simulink model "EMT"  (R2024b)
settings: Solver=ode5  StartTime=0.0  StopTime=1500  FixedStep=0.002  RelTol=1e-3
PreLoadFcn:
  | parameter;
InitFcn:
  | parameter;
StopFcn:
  | save('result.mat');
values from neighbouring files (symbols this model uses):
  A = 7.3    [parameter.m]
  a11 = (1+k1)*(1+k2)/k1/k2/iq    (= 1.54241568346)    [parameter.m]
  a11_L = a11    (= 1.54241568346)    [parameter.m]
  a12 = -(1+k1+k2)*(1+k3)/k1/k2    (= -3.86074191629)    [parameter.m]
  a12_L = a11*(1+k3+k4)/(1+k3)    (= 2.43173643789)    [parameter.m]
  a21 = -(1+k2)/k1/iq    (= -1.04963112005)    [parameter.m]
  a22 = (1+k1+k2)/k1    (= 2.46948356808)    [parameter.m]
  B = 2.71    [parameter.m]
  b11 = 0    [parameter.m]
  b12 = (1+k3)    (= 3.33)    [parameter.m]
  b21 = (1+k2)/iq    (= 2.23571428571)    [parameter.m]
  b22 = -k2    (= -2.13)    [parameter.m]
  C1_shift = 200    [parameter.m]
  Cb = 70    [parameter.m]
  Cd = 0.6    [parameter.m]
  eff_generator = eff_motor    [parameter.m]
  eff_motor = [0.80 0.80 0.84 0.84 0.83 0.85 0.83 0.83 0.83 0.80 0.80 0.80 ... (first row only)    [parameter.m]
  ele_map = [10.00,11.46,14.13,19.24,20.94,23.21,20.29,20.23,22.28,17.66,16.24,18.95,20.79,16.98,18.22,16.52,18.29,20.67,20.82,23.14,23.36,21.30,17.71,20.26,19.53,21.18,23.13,22.79,19.35,16.77,20.50,19.02,20.56,21.90,23.91,20.40,18.45,22.70,22.38,22.48,21.84,17.76,20.13,22.61,19.35,19.36,21.56,20.37,18.38,17.96,18.38,17.24,18.99,22.31,23.50,18.24,22.11,20.73,20.35,18.91,22.88,20.92,18.75,16.85,21.94,17.80,19. ...(+2007 chars)    [parameter.m]
  Fb_max = 5.5*mass    (= 247500)    [parameter.m]
  ic = 4.42    [parameter.m]
  JA = 0.4    [parameter.m]
  JB = JA    (= 0.4)    [parameter.m]
  Jc3r4 = 1e-2    (= 0.01)    [parameter.m]
  Je = 2.5    [parameter.m]
  Jh = 1e-2    (= 0.01)    [parameter.m]
  kh = 2.88    [parameter.m]
  kt = 1.83    [parameter.m]
  L = 4.472    [parameter.m]
  mass = 45000    [parameter.m]
  miu_max = 0.8    [parameter.m]
  n_generator = n_motor    [parameter.m]
  n_motor = [0 0.1 0.25 0.4 0.55 0.7 0.85 1 1.15 1.3 1.45 2.2]*3185    [parameter.m]
  nA_map = [-6000:50:-3250 -3200 0 3200 3250:50:6000]    [parameter.m]    (also in plot_result.m = [-7000:50:-3250 -3200 0 3200 3250:50:7000])
  nA_max = max(nA_map)    [parameter.m]
  nA_min = min(nA_map)    [parameter.m]
  nB_map = nA_map    [parameter.m]    (also in plot_result.m = [-7000:50:-3250 -3200 0 3200 3250:50:7000])
  nB_max = nA_max    [parameter.m]
  nB_min = nA_min    [parameter.m]
  ne_idl = 3000    [parameter.m]
  ne_map = [1600,1700,1800,1900,2000,2100,2200,2300,2400,2500,2600,2700,2800,2900,3000,3100,3200,3300,3400,3500,3600,3700,3800,3900,4000,4100,4200,4500]    [parameter.m]
  ne_max = 4200    [parameter.m]
  ne_min = 1600    [parameter.m]
  ne_start = 200    [parameter.m]
  nZ_map = [-8000:50:-4850 -4800 0 4800 4850:50:8000]    [parameter.m]
  Pb_epr = [-45 -45 -40 -30 0 30 40 45 45]    [parameter.m]
  Pb_max = [0 40 45 45 45]    [parameter.m]
  Pb_min = [-45 -45 -45 -40 0]    [parameter.m]
  Pe_ass = 210+20    (= 230)    [parameter.m]
  Pe_max = 1103    [parameter.m]
  PN0 = 0    [parameter.m]
  R_map = [0.90 0.89 0.90 0.91 0.92 0.93 0.94 0.95 0.96 0.97 0.98]/10    [parameter.m]
  rz = 0.318    [parameter.m]
  SOC0 = 60    [parameter.m]
  SOC_epr = [30 31 50 59 60 61 70 79 80]    [parameter.m]
  SOC_map = 0:10:100    [parameter.m]
  T_generator = T_motor    [parameter.m]
  T_motor = [0 0.3 0.8 1.3 1.8 2.3 2.8]/1.8*1110    [parameter.m]
  TA_max_map = [370*9549./(6000:-50:3250) 1110 1110 1110 370*9549./(3250:50:6000)]    [parameter.m]    (also in plot_result.m = [370*9549./(7000:-50:3250) 1100 1100 1100 370*9549./(3250:50)
  TA_min_map = -TA_max_map    [parameter.m]
  TAf = 0    [parameter.m]
  TB_max_map = TA_max_map    [parameter.m]    (also in plot_result.m = [370*9549./(7000:-50:3250) 1110 1110 1110 370*9549./(3250:50)
  TB_min_map = TA_min_map    [parameter.m]
  TBf = TAf    (= 0)    [parameter.m]
  Te_map = [0,599,798,998,1168,1324,1495,1660,1822,1970,2106,2235,2355,2458,2508,2543,2565,2606,2613,2649,2658,2689,2701,2707,2719,2724,2728,2740,2743,2754]    [parameter.m]
  Te_max_map = [1168,1324,1495,1660,1822,1970,2106,2235,2355,2458,2543,2606,2658,2701,2728,2743,2754,2743,2740,2724,2719,2707,2689,2649,2613,2565,2508,998]    [parameter.m]
  Te_start = 1600    [parameter.m]
  Tef = 100    [parameter.m]
  Time = 0:0.1:200    [parameter.m]
  Time_ele = 0:4:1600    [parameter.m]
  TS_A = 0.2    [parameter.m]
  TS_B = TS_A    (= 0.2)    [parameter.m]
  TS_C0 = 0.2    [parameter.m]
  TS_C1 = 0.2    [parameter.m]
  Ts_e = 0.1    [parameter.m]
  TS_Z1 = 0.2    [parameter.m]
  TS_Z2 = 0.2    [parameter.m]
  TZ_max_map = [450*9549./(8000:-50:4850) 1000 1000 1000 450*9549./(4850:50:8000)]    [parameter.m]
  TZ_min_map = -TZ_max_map    [parameter.m]
  Uoc_map = [3.258,3.668,3.733,3.783,3.833,3.877,3.912,3.941,3.973,4.013,4.200]*250    [parameter.m]
  v_cyc = 0.*(0<=Time&Time<11)+(3.75.*Time-41.25).*(11<=Time&Time<15)+15.*(15<=Time&Time<23)+(-3.*Time+84).*(23<=Time&Time<28)+0.*(28<=Time&Time<49)+(8.*Time/3-392/3).*(49<=Time&Time<61)+32.*(61<=Time&Time<85)+(-32.*Time/11+3072/11).*(85<=Time&Time<96)+0.*(96<=Time&Time<117)+(25.*Time/13-2925/13).*(117<=Time&Time<143)+50.*(143<=Time&Time<155)+(-15.*Time/8+2725/8).*(155<=Time&Time<163)+35.*(163<=Time&Time<17 ...(+70 chars)    [parameter.m]
  V_Shift12 = 32    [parameter.m]
  V_Shift21 = 25    [parameter.m]
  Voltage_epr = [750 760 900 1000 1050]    [parameter.m]
  Y_engine = 0.955    [parameter.m]
  Yc = 0.98    [parameter.m]
  Yh = 0.96    [parameter.m]
  Z1_shift = 200    [parameter.m]
  Z2_shift = 200    [parameter.m]
undefined symbols (not defined in the file or in its folder): sigbuilder_block
libraries: fl_lib x82, nesl_utility x55, simulink x49, sdl_lib x10, simulink_need_slupdate x6, powerlib_extras x1
(part 2 of 6)

== system EMT/Control Unit/Control/Stage Judge ==
  Add : Sum  Inputs=++++
  EVT1_H Stage : Subsystem
  EVT2 Stage : Subsystem
  Prepare Stage : Subsystem
  Shift Stage : Subsystem
  stage : Outport
  tag scope: stage=global
  wires:
  EVT2 Stage/1(Out1) -> Add/4
  EVT1_H Stage/1(Out1) -> Add/2
  Shift Stage/1(Out1) -> Add/3
  Prepare Stage/1(Out1) -> Add/1
  Add/1 -> stage/1, [stage]

== system EMT/Control Unit/Driver/Electric Power Requirement ==
  " 0.1" : ManualSwitch  CurrentSetting=0
  1-D Lookup Table1 : Lookup_n-D  NumberOfTableDimensions=1  BreakpointsForDimension1=Time_ele  Table=ele_map  RndMeth=Simplest
  10 : ManualSwitch
  Add Power : ManualSwitch
  Clock1 : Clock
  ElectricPower : Display
  Saturation : Saturate  UpperLimit=300  LowerLimit=0
  Sub Power : ManualSwitch  CurrentSetting=0
  Subsystem4 : Subsystem  mask{Parameter1=on}
      mask prompts: Parameter1 "Pedal"
  Subsystem6 : Subsystem
  Transfer Fcn1 : TransferFcn  Denominator=[0.02 1]
  tag scope: ElectricPower=global
  wires:
  Subsystem4/1(Out1) -> Add Power/1
  Subsystem4/2(Out2) -> Add Power/2
  Subsystem4/3(Out3) -> Sub Power/1
  Add Power/1 -> Subsystem6/1(Add)
  Sub Power/1 -> Subsystem6/2(Sub)
  Subsystem4/4(Out4) -> Sub Power/2
  Subsystem4/5(Out5) -> " 0.1"/1
  Subsystem4/6(Out6) -> " 0.1"/2
  Subsystem4/7(Out7) -> 10/1
  Subsystem4/8(Out8) -> 10/2
  " 0.1"/1 -> Subsystem6/3(0.1)
  10/1 -> Subsystem6/4(10)
  Clock1/1 -> 1-D Lookup Table1/1
  Transfer Fcn1/1 -> [ElectricPower], ElectricPower/1
  Saturation/1 -> Transfer Fcn1/1
  1-D Lookup Table1/1 -> Saturation/1

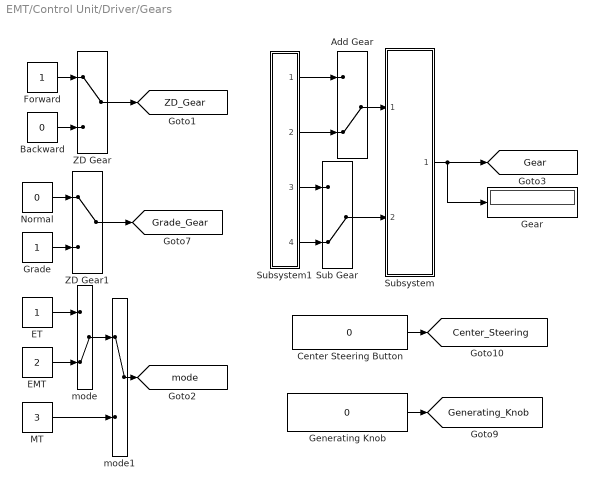
== system EMT/Control Unit/Driver/Gears ==
  "Add Gear " : ManualSwitch  CurrentSetting=0
  Backward : Constant  Value=0
  Center Steering Button : Constant  Value=0
  EMT : Constant  Value=2
  ET : Constant
  Forward : Constant
  Gear : Display
  Generating Knob : Constant  Value=0
  Grade : Constant
  MT : Constant  Value=3
  Normal : Constant  Value=0
  Sub Gear : ManualSwitch  CurrentSetting=0
  Subsystem : Subsystem
  Subsystem1 : Subsystem
  ZD Gear : ManualSwitch
  ZD Gear1 : ManualSwitch
  mode : ManualSwitch  CurrentSetting=0
  mode1 : ManualSwitch
  tag scope: Center_Steering=global, Gear=global, Generating_Knob=global, Grade_Gear=global, ZD_Gear=global, mode=global
  wires:
  ZD Gear1/1 -> [Grade_Gear]
  Normal/1 -> ZD Gear1/1
  Grade/1 -> ZD Gear1/2
  Center Steering Button/1 -> [Center_Steering]
  Generating Knob/1 -> [Generating_Knob]
  mode/1 -> mode1/1
  mode1/1 -> [mode]
  MT/1 -> mode1/2
  EMT/1 -> mode/2
  Subsystem/1(Gear) -> [Gear], Gear/1
  Sub Gear/1 -> Subsystem/2(Sub)
  "Add Gear "/1 -> Subsystem/1(Add)
  Subsystem1/4(4) -> Sub Gear/2
  Subsystem1/3(3) -> Sub Gear/1
  Subsystem1/2(2) -> "Add Gear "/2
  Subsystem1/1(1) -> "Add Gear "/1
  ET/1 -> mode/1
  ZD Gear/1 -> [ZD_Gear]
  Forward/1 -> ZD Gear/1
  Backward/1 -> ZD Gear/2

== system EMT/Control Unit/Driver/Grade Angle ==
  " 0.1" : ManualSwitch  CurrentSetting=0
  10 : ManualSwitch
  Add angle : ManualSwitch
  Forward : Constant  Value=32
  Forward1 : Constant  Value=0
  Sub angle : ManualSwitch  CurrentSetting=0
  Subsystem4 : Subsystem  mask{Parameter1=on}
      mask prompts: Parameter1 "Pedal"
  Subsystem6 : Subsystem
  Transfer Fcn1 : TransferFcn  Denominator=[0.02 1]
  angle : Display
  tag scope: angle=global
  wires:
  Subsystem4/1(Out1) -> Add angle/1
  Subsystem4/2(Out2) -> Add angle/2
  Subsystem4/3(Out3) -> Sub angle/1
  Add angle/1 -> Subsystem6/1(Add)
  Sub angle/1 -> Subsystem6/2(Sub)
  Subsystem4/4(Out4) -> Sub angle/2
  Subsystem4/5(Out5) -> " 0.1"/1
  Subsystem4/6(Out6) -> " 0.1"/2
  Subsystem4/7(Out7) -> 10/1
  Subsystem4/8(Out8) -> 10/2
  " 0.1"/1 -> Subsystem6/3(0.1)
  10/1 -> Subsystem6/4(10)
  Subsystem6/1(angle) -> Transfer Fcn1/1, angle/1
  Forward1/1 -> [angle]

== system EMT/Control Unit/Driver/Ground Resistance Coefficient ==
  *0.1 : ManualSwitch
  *10 : ManualSwitch
  Add : Sum
  Add fg : ManualSwitch  CurrentSetting=0
  Add1 : Sum
  Forward : Constant  Value=0.07
  Forward1 : Constant  Value=0.045
  Road : Subsystem
  Road1 : Subsystem
  Saturation : Saturate  UpperLimit=0.6  LowerLimit=0.04
  Saturation1 : Saturate  UpperLimit=0.6  LowerLimit=0.04
  Sub fg : ManualSwitch  CurrentSetting=0
  Subsystem2 : Subsystem  mask{Parameter1=on}
      mask prompts: Parameter1 "Pedal"
  Subsystem3 : Subsystem
  Transfer Fcn1 : TransferFcn  Denominator=[0.02 1]
  Uniform Random Number : UniformRandomNumber  Minimum=-0.01  Maximum=0.01  SampleTime=1
  fg : Display
  tag scope: fg_act=global
  wires:
  Road/1(fg) -> Add/2
  Subsystem3/1(fg) -> Add/1
  Subsystem2/1(Out1) -> Add fg/1
  Subsystem2/2(Out2) -> Add fg/2
  Subsystem2/3(Out3) -> Sub fg/1
  Add fg/1 -> Subsystem3/1(Add)
  Sub fg/1 -> Subsystem3/2(Sub)
  Subsystem2/4(Out4) -> Sub fg/2
  Subsystem2/5(Out5) -> *0.1/1
  Subsystem2/6(Out6) -> *0.1/2
  Subsystem2/7(Out7) -> *10/1
  Subsystem2/8(Out8) -> *10/2
  *0.1/1 -> Subsystem3/3(0.1)
  *10/1 -> Subsystem3/4(10)
  Transfer Fcn1/1 -> fg/1
  Add/1 -> Saturation/1
  Uniform Random Number/1 -> Add1/2
  Road1/1(fg) -> Saturation1/1
  Forward/1 -> Add1/1
  Add1/1 -> Transfer Fcn1/1
  Forward1/1 -> [fg_act]

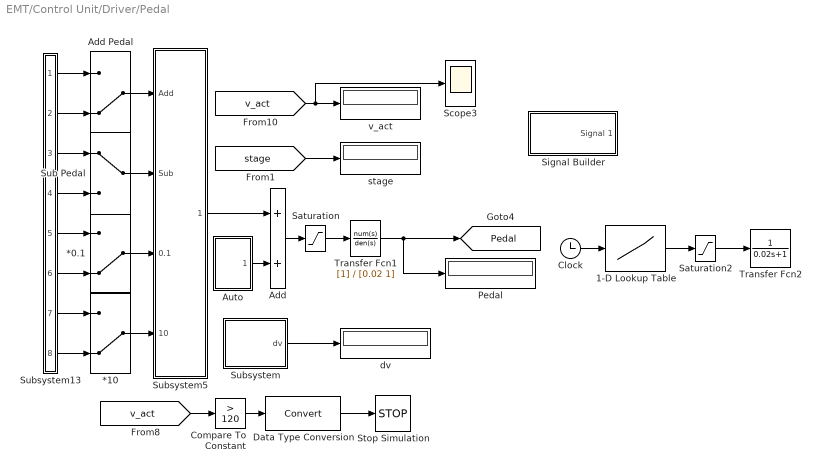
== system EMT/Control Unit/Driver/Pedal  ==
  *0.1 : ManualSwitch  CurrentSetting=0
  *10 : ManualSwitch  CurrentSetting=0
  1-D Lookup Table : Lookup_n-D  NumberOfTableDimensions=1  BreakpointsForDimension1=[0 100 101 200]  Table=[1 1 -1 -1]  RndMeth=Simplest
  Add : Sum
  Add Pedal : ManualSwitch  CurrentSetting=0
  Auto : Subsystem
  Clock : Clock
  Compare To Constant : simulink/Logic and Bit Operations/Compare To Constant  relop=>  const=120  OutDataTypeStr=uint8
  Data Type Conversion : DataTypeConversion  SaturateOnIntegerOverflow=off  RndMeth=Floor
  Pedal : Display
  Saturation : Saturate  UpperLimit=1  LowerLimit=-1
  Saturation2 : Saturate  UpperLimit=1  LowerLimit=-1
  Scope3 : Scope
  Signal Builder : Subsystem  Tag=STV Subsys  LoadFcn=sigbuilder_block('load');  StartFcn=sigbuilder_block('start');  StopFcn=sigbuilder_block('stop');  ClipboardFcn=sigbuilder_block('clipboard');  mask(Sigbuilder block){tuvar=[0:10]}
      mask help: Simulink:masks:SigbuilderBlock_MD
      mask init:
      | if ~strcmp(get_param(bdroot(gcbh),'SimulationStatus'),'stopped') tuvar = sigbuilder_block('maskInit'); end
      settings: CopyFcn=sigbuilder_block('copy');  DeleteFcn=sigbuilder_block('delete');  ModelCloseFcn=sigbuilder_block('modelClose');  PreSaveFcn=sigbuilder_block('preSave');  PauseFcn=sigbuilder_block('pause')  ContinueFcn=sigbuilder_block('continue')  NameChangeFcn=sigbuilder_block('namechange');  OpenFcn=sigbuilder_block('open',[437.25 199.5 550.5 399.75 ]);  CloseFcn=sigbuilder_block('close');
      mask Display: plot(0, 0, 100, 100,[2, 2, 32, 32, 2], [68, 8, 8, 68, 68],[32, 2], [38, 38], [32, 19, 2],[53, 60, 44], [32, 17, 17, 2],[16, 16, 31, 31]);txt = getActiveGroup(gcbh);text(2, 100, txt,'verticalAlignment', 'top');
  Stop Simulation : Stop
  Sub Pedal : ManualSwitch
  Subsystem : Subsystem
  Subsystem13 : Subsystem  mask{Parameter1=on}
      mask prompts: Parameter1 "Pedal"
  Subsystem5 : Subsystem
  Transfer Fcn1 : TransferFcn  Denominator=[0.02 1]
  Transfer Fcn2 : TransferFcn  Denominator=[0.02 1]
  dv : Display
  stage : Display
  v_act : Display
  tag scope: Pedal=global
  wires:
  Subsystem5/1(Pedal) -> Add/1
  Subsystem/1(dv) -> dv/1
  [stage] -> stage/1
  [v_act] -> Scope3/1, v_act/1
  *10/1 -> Subsystem5/4(10)
  *0.1/1 -> Subsystem5/3(0.1)
  Subsystem13/8(Out8) -> *10/2
  Subsystem13/7(Out7) -> *10/1
  Subsystem13/6(Out6) -> *0.1/2
  Subsystem13/5(Out5) -> *0.1/1
  Subsystem13/4(Out4) -> Sub Pedal/2
  Sub Pedal/1 -> Subsystem5/2(Sub)
  Add Pedal/1 -> Subsystem5/1(Add)
  Subsystem13/3(Out3) -> Sub Pedal/1
  Subsystem13/2(Out2) -> Add Pedal/2
  Subsystem13/1(Out1) -> Add Pedal/1
  [v_act] -> Compare To Constant/1
  Compare To Constant/1 -> Data Type Conversion/1
  Data Type Conversion/1 -> Stop Simulation/1
  Saturation/1 -> Transfer Fcn1/1
  Add/1 -> Saturation/1
  Clock/1 -> 1-D Lookup Table/1
  1-D Lookup Table/1 -> Saturation2/1
  Saturation2/1 -> Transfer Fcn2/1
  Auto/1(Pedal) -> Add/2
  Transfer Fcn1/1 -> Pedal/1, [Pedal]

== system EMT/Control Unit/Driver/Wheel Angle ==
  " x 0.1" : ManualSwitch  CurrentSetting=0
  Add wheel : ManualSwitch
  Sub Wheel : ManualSwitch  CurrentSetting=0
  Subsystem1 : Subsystem  mask{Parameter1=on}
      mask prompts: Parameter1 "Pedal"
  Subsystem2 : Subsystem
  Wheel : Display
  x10 : ManualSwitch
  tag scope: Wheel=global
  wires:
  Subsystem2/1(wheel) -> Wheel/1, [Wheel]
  Subsystem1/1(Out1) -> Add wheel/1
  Subsystem1/2(Out2) -> Add wheel/2
  Subsystem1/3(Out3) -> Sub Wheel/1
  Add wheel/1 -> Subsystem2/1(Add)
  Sub Wheel/1 -> Subsystem2/2(Sub)
  Subsystem1/4(Out4) -> Sub Wheel/2
  Subsystem1/5(Out5) -> " x 0.1"/1
  Subsystem1/6(Out6) -> " x 0.1"/2
  Subsystem1/7(Out7) -> x10/1
  Subsystem1/8(Out8) -> x10/2
  " x 0.1"/1 -> Subsystem2/3(0.1)
  x10/1 -> Subsystem2/4(10)

== system EMT/Front Gear/C0/C0 ==
  Press : Inport
  C0 : sdl_lib/Clutches/Disc Friction Clutch  geometry_model=2  r_eff=130 mm  d_o=145*2 mm  d_i=110*2 mm  nS=6  piston_area=0.0347 m^2  unidirectional=0  friction_model=1  mu_w_vector=[ 0 0.1 0.2 0.3 0.4 0.5 1 2 5 10 100 1000 ] rad/s  temperature_TLU=[280.0, 300.0, 320.0] K  mu_static=0.10  mu_static_vector=[0.4, 0.38, 0.36]  mu_coulomb=0.06  mu_coulomb_vector=[ 0.29 0.28 0.26 0.22 0.21 0.2 0.2 0.19 0.19 0.19 0.19 0.19 ]  mu_coulomb_temp_vector=[0.3, 0.28, 0.25]  mu_coulomb_matrix=[0.34, 0.32, 0.3; 0.3, 0.28, 0.25; 0.25, 0.2, 0.15]  mu_interp_method=1  mu_extrap_method=1  d_f=0.6  w_tol=0.001 rad/s  pressure_min=1560 Pa  mu_visc=0.0256 N*m/(rad/s)  initial_state_locked=1  thermal_mass=25 kJ/K  T_init=300 K
      settings: InternalSimscapePortConfiguration="{\"Bottom\":[],\"Left\":[{\"id\":\"P\",\"label\":\"P\",\"type\":\"input\"},{\"id\":\"B\",\"label\":\"B\",\"type\":\"foundation.mechanical.rotational.rotational\"}],\"Right\":[{\"id\":\"F\",\"label\":\"F\",\"type\":\"foundation.mechanical.rotational.rotational\"}],\"Top\":[]}"
  Simulink-PS Converter : nesl_utility/Simulink-PS Converter  PhysicalDomain=network_engine_domain  SubClassName=ps_input  LeftPortType=input  RightPortType=output  PseudoPeriodic=off  Frequencies=[]  NoiseDistribution=none  NoiseParameters=[]  Unit=Pa  AffineConversion=off  FilteringAndDerivatives=filter  SimscapeFilterOrder=1  InputFilterTimeConstant=.001  UdotUserProvided=1
  Slip Sensor : Subsystem  mask(Slip Sensor){}
      mask help: The speed unit is r/min.
  Tire Radius2 : Gain  Gain=2500000
  In : PMIOPort  Side=Left
  Out : PMIOPort  Port=2  Side=Right
  r/min : Outport
  wires:
  Slip Sensor/1(r/min) -> r/min/1
  Press/1 -> Tire Radius2/1
  Tire Radius2/1 -> Simulink-PS Converter/1
  connections:
  Slip Sensor/LConn1 -- C0/LConn2 -- In/RConn1
  Slip Sensor/RConn1 -- C0/RConn1 -- Out/RConn1
  Simulink-PS Converter/RConn1 -- C0/LConn1

== system EMT/Front Gear/C0/Power ==
  Gain1 : Gain  Gain=1/9549
  Product3 : Product  RndMeth=Zero
  Speed Sensor : Subsystem  mask(Speed Sensor){}
      mask help: The speed unit is r/min.
  Torque Sensor : Subsystem  mask(Torque Sensor){}
      mask help: The torque unit is Nm.
  In : PMIOPort  Side=Left
  Out : PMIOPort  Port=2  Side=Right
  kW : Outport
  wires:
  Speed Sensor/1(r/min) -> Product3/2
  Torque Sensor/1(Nm) -> Gain1/1
  Gain1/1 -> Product3/1
  Product3/1 -> kW/1
  connections:
  Out/RConn1 -- Torque Sensor/RConn1 -- Speed Sensor/LConn1
  In/RConn1 -- Torque Sensor/LConn1

== system EMT/Front Gear/C0/Power1 ==
  Gain1 : Gain  Gain=1/9549
  Product3 : Product  RndMeth=Zero
  Speed Sensor : Subsystem  mask(Speed Sensor){}
      mask help: The speed unit is r/min.
  Torque Sensor : Subsystem  mask(Torque Sensor){}
      mask help: The torque unit is Nm.
  In : PMIOPort  Side=Left
  Out : PMIOPort  Port=2  Side=Right
  kW : Outport
  wires:
  Product3/1 -> kW/1
  Gain1/1 -> Product3/1
  Torque Sensor/1(Nm) -> Gain1/1
  Speed Sensor/1(r/min) -> Product3/2
  connections:
  In/RConn1 -- Torque Sensor/LConn1
  Torque Sensor/RConn1 -- Out/RConn1 -- Speed Sensor/LConn1

== system EMT/Front Gear/Subsystem/Speed Sensor ==
  Ideal Rotational Motion Sensor : fl_lib/Mechanical/Mechanical Sensors/Ideal Rotational Motion Sensor  reference=foundation.enum.MeasurementReference.difference  acceleration_port=false  velocity_port=true  position_port=true  wrap_angle=false  offset=0 rad
  PS-Simulink Converter : nesl_utility/PS-Simulink Converter  PhysicalDomain=network_engine_domain  SubClassName=ps_output  LeftPortType=input  RightPortType=output  PseudoPeriodic=off  Frequencies=[]  VectorFormat=1-D array  Unit=rad/s  AffineConversion=off
  Reference : fl_lib/Mechanical/Rotational Elements/Mechanical Rotational Reference
  Tire Radius2 : Gain  Gain=30/pi
  shaft : PMIOPort  Side=Left
  r/min : Outport
  wires:
  Tire Radius2/1 -> r/min/1
  PS-Simulink Converter/1 -> Tire Radius2/1
  connections:
  shaft/RConn1 -- Ideal Rotational Motion Sensor/LConn1
  Reference/LConn1 -- Ideal Rotational Motion Sensor/RConn1
  PS-Simulink Converter/LConn1 -- Ideal Rotational Motion Sensor/RConn2

== system EMT/Front Gear/Subsystem/Torque Sensor ==
  Ideal Torque Sensor : fl_lib/Mechanical/Mechanical Sensors/Ideal Torque Sensor
  PS-Simulink Converter : nesl_utility/PS-Simulink Converter  PhysicalDomain=network_engine_domain  SubClassName=ps_output  LeftPortType=input  RightPortType=output  PseudoPeriodic=off  Frequencies=[]  VectorFormat=1-D array  Unit=1  AffineConversion=off
  In : PMIOPort  Side=Left
  Out : PMIOPort  Port=2  Side=Right
  Nm : Outport
  wires:
  PS-Simulink Converter/1 -> Nm/1
  connections:
  PS-Simulink Converter/LConn1 -- Ideal Torque Sensor/RConn2
  In/RConn1 -- Ideal Torque Sensor/LConn1
  Ideal Torque Sensor/RConn1 -- Out/RConn1

== system EMT/Power Coupler /C1/C2 ==
  Press : Inport
  C1 : sdl_lib/Clutches/Disc Friction Clutch  geometry_model=2  r_eff=130 mm  d_o=167*2 mm  d_i=143*2 mm  nS=8  piston_area=0.0290 m^2  unidirectional=0  friction_model=1  mu_w_vector=[ 0 0.1 0.2 0.3 0.4 0.5 1 2 5 10 100 1000 ] rad/s  temperature_TLU=[280.0, 300.0, 320.0] K  mu_static=0.10  mu_static_vector=[0.4, 0.38, 0.36]  mu_coulomb=0.06  mu_coulomb_vector=[ 0.29 0.28 0.26 0.22 0.21 0.2 0.2 0.19 0.19 0.19 0.19 0.19 ]  mu_coulomb_temp_vector=[0.3, 0.28, 0.25]  mu_coulomb_matrix=[0.34, 0.32, 0.3; 0.3, 0.28, 0.25; 0.25, 0.2, 0.15]  mu_interp_method=1  mu_extrap_method=1  d_f=0.6  w_tol=0.001 rad/s  pressure_min=1840 Pa  mu_visc=0.0414 N*m/(rad/s)  initial_state_locked=0  thermal_mass=25 kJ/K  T_init=300 K
      settings: InternalSimscapePortConfiguration="{\"Bottom\":[],\"Left\":[{\"id\":\"P\",\"label\":\"P\",\"type\":\"input\"},{\"id\":\"B\",\"label\":\"B\",\"type\":\"foundation.mechanical.rotational.rotational\"}],\"Right\":[{\"id\":\"F\",\"label\":\"F\",\"type\":\"foundation.mechanical.rotational.rotational\"}],\"Top\":[]}"
  Simulink-PS Converter : nesl_utility/Simulink-PS Converter  PhysicalDomain=network_engine_domain  SubClassName=ps_input  LeftPortType=input  RightPortType=output  PseudoPeriodic=off  Frequencies=[]  NoiseDistribution=none  NoiseParameters=[]  Unit=Pa  AffineConversion=off  FilteringAndDerivatives=filter  SimscapeFilterOrder=1  InputFilterTimeConstant=.001  UdotUserProvided=1
  Slip Sensor : Subsystem  mask(Slip Sensor){}
      mask help: The speed unit is r/min.
  Tire Radius2 : Gain  Gain=2500000
  In : PMIOPort  Side=Left
  Out : PMIOPort  Port=2  Side=Right
  r/min : Outport
  wires:
  Tire Radius2/1 -> Simulink-PS Converter/1
  Press/1 -> Tire Radius2/1
  Slip Sensor/1(r/min) -> r/min/1
  connections:
  Simulink-PS Converter/RConn1 -- C1/LConn1
  In/RConn1 -- C1/LConn2 -- Slip Sensor/LConn1
  C1/RConn1 -- Out/RConn1 -- Slip Sensor/RConn1

== system EMT/Power Coupler /C1/Power ==
  Gain1 : Gain  Gain=1/9549
  Product3 : Product  RndMeth=Zero
  Speed Sensor : Subsystem  mask(Speed Sensor){}
      mask help: The speed unit is r/min.
  Torque Sensor : Subsystem  mask(Torque Sensor){}
      mask help: The torque unit is Nm.
  In : PMIOPort  Side=Left
  Out : PMIOPort  Port=2  Side=Right
  kW : Outport
  wires:
  Product3/1 -> kW/1
  Gain1/1 -> Product3/1
  Torque Sensor/1(Nm) -> Gain1/1
  Speed Sensor/1(r/min) -> Product3/2
  connections:
  In/RConn1 -- Torque Sensor/LConn1
  Torque Sensor/RConn1 -- Out/RConn1 -- Speed Sensor/LConn1

== system EMT/Power Coupler /C1/Power1 ==
  Gain1 : Gain  Gain=1/9549
  Product3 : Product  RndMeth=Zero
  Speed Sensor : Subsystem  mask(Speed Sensor){}
      mask help: The speed unit is r/min.
  Torque Sensor : Subsystem  mask(Torque Sensor){}
      mask help: The torque unit is Nm.
  In : PMIOPort  Side=Left
  Out : PMIOPort  Port=2  Side=Right
  kW : Outport
  wires:
  Speed Sensor/1(r/min) -> Product3/2
  Torque Sensor/1(Nm) -> Gain1/1
  Gain1/1 -> Product3/1
  Product3/1 -> kW/1
  connections:
  Speed Sensor/LConn1 -- Out/RConn1 -- Torque Sensor/RConn1
  In/RConn1 -- Torque Sensor/LConn1

== system EMT/Power Coupler /Z1/Z ==
  Abs : Abs  SaturateOnIntegerOverflow=off
  Add : Sum  Inputs=+-
  Power : Subsystem
  Power1 : Subsystem
  Z1 : Subsystem
  In : PMIOPort  Side=Left
  Out : PMIOPort  Port=2  Side=Right
  tag scope: Z1_loss=global, Z1_rela=global
  wires:
  Z1/1(r/min) -> [Z1_rela]
  [Press_Z1] -> Z1/1(Press)
  Power1/1(kW) -> Add/2
  Power/1(kW) -> Add/1
  Abs/1 -> [Z1_loss]
  Add/1 -> Abs/1
  connections:
  In/RConn1 -- Power/LConn1
  Power/RConn1 -- Z1/LConn1
  Z1/RConn1 -- Power1/LConn1
  Power1/RConn1 -- Out/RConn1

== system EMT/Power Coupler /Z2/Z ==
  Abs : Abs  SaturateOnIntegerOverflow=off
  Add : Sum  Inputs=+-
  Power : Subsystem
  Power1 : Subsystem
  Z2 : Subsystem
  In : PMIOPort  Side=Left
  Out : PMIOPort  Port=2  Side=Right
  tag scope: Z2_loss=global, Z2_rela=global
  wires:
  [Press_Z2] -> Z2/1(Press)
  Z2/1(r/min) -> [Z2_rela]
  Add/1 -> Abs/1
  Abs/1 -> [Z2_loss]
  Power1/1(kW) -> Add/2
  Power/1(kW) -> Add/1
  connections:
  In/RConn1 -- Power/LConn1
  Power/RConn1 -- Z2/LConn1
  Z2/RConn1 -- Power1/LConn1
  Power1/RConn1 -- Out/RConn1

== system EMT/Rear Gear/Subsystem/Speed Sensor ==
  Ideal Rotational Motion Sensor : fl_lib/Mechanical/Mechanical Sensors/Ideal Rotational Motion Sensor  reference=foundation.enum.MeasurementReference.difference  acceleration_port=false  velocity_port=true  position_port=true  wrap_angle=false  offset=0 rad
  PS-Simulink Converter : nesl_utility/PS-Simulink Converter  PhysicalDomain=network_engine_domain  SubClassName=ps_output  LeftPortType=input  RightPortType=output  PseudoPeriodic=off  Frequencies=[]  VectorFormat=1-D array  Unit=rad/s  AffineConversion=off
  Reference : fl_lib/Mechanical/Rotational Elements/Mechanical Rotational Reference
  Tire Radius2 : Gain  Gain=30/pi
  shaft : PMIOPort  Side=Left
  r/min : Outport
  wires:
  Tire Radius2/1 -> r/min/1
  PS-Simulink Converter/1 -> Tire Radius2/1
  connections:
  shaft/RConn1 -- Ideal Rotational Motion Sensor/LConn1
  Reference/LConn1 -- Ideal Rotational Motion Sensor/RConn1
  PS-Simulink Converter/LConn1 -- Ideal Rotational Motion Sensor/RConn2

== system EMT/Rear Gear/Subsystem/Torque Sensor ==
  Ideal Torque Sensor : fl_lib/Mechanical/Mechanical Sensors/Ideal Torque Sensor
  PS-Simulink Converter : nesl_utility/PS-Simulink Converter  PhysicalDomain=network_engine_domain  SubClassName=ps_output  LeftPortType=input  RightPortType=output  PseudoPeriodic=off  Frequencies=[]  VectorFormat=1-D array  Unit=1  AffineConversion=off
  In : PMIOPort  Side=Left
  Out : PMIOPort  Port=2  Side=Right
  Nm : Outport
  wires:
  PS-Simulink Converter/1 -> Nm/1
  connections:
  PS-Simulink Converter/LConn1 -- Ideal Torque Sensor/RConn2
  In/RConn1 -- Ideal Torque Sensor/LConn1
  Ideal Torque Sensor/RConn1 -- Out/RConn1

== system EMT/Simulation Results/Engine Viewer/Fuel  ==
  FuelConsumption : Lookup2D  RowIndex=ne_map  ColumnIndex=Te_map  Table=fuel_map'  LookUpMeth=Interpolation-Use End Values  SaturateOnIntegerOverflow=off  InputSameDT=off
  Gain : Gain  Gain=1/3600/0.84/1000
  Gain1 : Gain  Gain=1/9549
  Integrator : Integrator  IgnoreLimit=on
  Product1 : Product  RndMeth=Zero
  Product2 : Product  RndMeth=Zero
  Product3 : Product  RndMeth=Zero
  Saturation : Saturate  UpperLimit=max(ne_map)  LowerLimit=min(ne_map)
  Saturation1 : Saturate  UpperLimit=max(Te_map)  LowerLimit=min(Te_map)
  Saturation2 : Saturate  UpperLimit=max(ne_map)*max(Te_map)/9549  LowerLimit=0
  fuel_L : Outport
  gpkWh : Outport  Port=2
  tag scope: eng_fuel_gpkWh=global, fuel_L=global
  wires:
  [Te_act] -> Product1/2, Saturation1/1
  [ne_act] -> Product1/1, Saturation/1
  Saturation2/1 -> Product3/2
  Gain1/1 -> Saturation2/1
  Saturation1/1 -> FuelConsumption/2
  Gain/1 -> Integrator/1
  Integrator/1 -> [fuel_L], fuel_L/1
  Product3/1 -> Gain/1
  Saturation/1 -> FuelConsumption/1
  Product1/1 -> Gain1/1
  Product2/1 -> Product3/1, [eng_fuel_gpkWh], gpkWh/1
  [engine_switch] -> Product2/1
  FuelConsumption/1 -> Product2/2

== system EMT/Simulation Results/Vehicle Viewer/Subsystem1 ==
  0 : Inport
  Constant : Constant  Value=0.001
  MinMax : MinMax  Function=max  Inputs=2
  1 : Outport
  wires:
  MinMax/1 -> 1/1
  0/1 -> MinMax/1
  Constant/1 -> MinMax/2

== system EMT/Simulation Results/Vehicle Viewer/Subsystem7 ==
  0 : Inport
  Constant : Constant  Value=0
  MinMax : MinMax  Function=max  Inputs=2
  1 : Outport
  wires:
  Constant/1 -> MinMax/2
  0/1 -> MinMax/1
  MinMax/1 -> 1/1

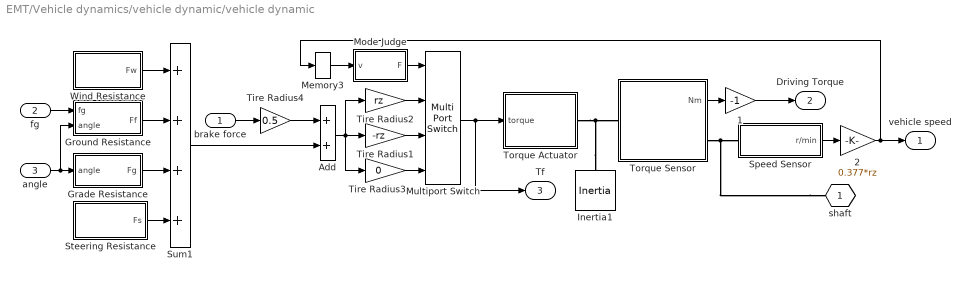
== system EMT/Vehicle dynamics/vehicle dynamic/vehicle dynamic ==
  brake force : Inport
  fg : Inport  Port=2
  angle : Inport  Port=3
  1 : Gain  Gain=-1
  2 : Gain  Gain=0.377*rz
  Add : Sum
  Grade Resistance : Subsystem
  Ground Resistance : Subsystem
  Inertia1 : fl_lib/Mechanical/Rotational Elements/Inertia  inertia=0.5*mass*rz^2 kg*m^2  num_ports=foundation.enum.numPorts2.one  w_specify=on  w_priority=High  w=0 rad/s  w_nominal_specify=off  w_nominal_value=1  w_nominal_unit=rad/s  t_specify=off  t_priority=None  t=0 N*m  t_nominal_specify=off  t_nominal_value=1  t_nominal_unit=N*m
  Memory3 : Memory
  Mode Judge : Subsystem
  Multiport Switch : MultiPortSwitch  SaturateOnIntegerOverflow=off  InputSameDT=off
  Speed Sensor : Subsystem  mask(Speed Sensor){}
      mask help: The speed unit is r/min.
  Steering Resistance : Subsystem
  Sum1 : Sum  Inputs=++++
  Tire Radius1 : Gain  Gain=-rz
  Tire Radius2 : Gain  Gain=rz
  Tire Radius3 : Gain  Gain=0
  Tire Radius4 : Gain  Gain=0.5
  Torque Actuator : Subsystem  mask(Torque Actuator){}
      mask help: The torque unit is Nm.
  Torque Sensor : Subsystem  mask(Torque Sensor){}
      mask help: The torque unit is Nm.
  Wind Resistance : Subsystem
  shaft : PMIOPort  Side=Left
  vehicle speed : Outport
  Driving Torque : Outport  Port=2
  Tf : Outport  Port=3
  wires:
  Tire Radius3/1 -> Multiport Switch/4
  Add/1 -> Tire Radius3/1, Tire Radius1/1, Tire Radius2/1
  Tire Radius1/1 -> Multiport Switch/3
  Tire Radius2/1 -> Multiport Switch/2
  Mode Judge/1(F) -> Multiport Switch/1
  1/1 -> Driving Torque/1
  Torque Sensor/1(Nm) -> 1/1
  Sum1/1 -> Add/2
  2/1 -> vehicle speed/1, Memory3/1
  brake force/1 -> Tire Radius4/1
  Speed Sensor/1(r/min) -> 2/1
  Ground Resistance/1(Ff) -> Sum1/2
  Wind Resistance/1(Fw) -> Sum1/1
  Tire Radius4/1 -> Add/1
  Steering Resistance/1(Fs) -> Sum1/4
  Grade Resistance/1(Fg) -> Sum1/3
  Memory3/1 -> Mode Judge/1(v)
  Multiport Switch/1 -> Torque Actuator/1(torque), Tf/1
  angle/1 -> Grade Resistance/1(angle), Ground Resistance/2(angle)
  fg/1 -> Ground Resistance/1(fg)
  connections:
  shaft/RConn1 -- Speed Sensor/LConn1 -- Torque Sensor/RConn1
  Inertia1/LConn1 -- Torque Actuator/RConn1 -- Torque Sensor/LConn1

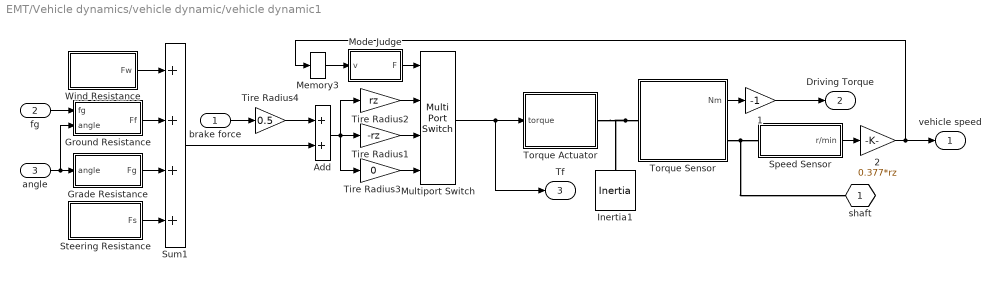
== system EMT/Vehicle dynamics/vehicle dynamic/vehicle dynamic1 ==
  brake force : Inport
  fg : Inport  Port=2
  angle : Inport  Port=3
  1 : Gain  Gain=-1
  2 : Gain  Gain=0.377*rz
  Add : Sum
  Grade Resistance : Subsystem
  Ground Resistance : Subsystem
  Inertia1 : fl_lib/Mechanical/Rotational Elements/Inertia  inertia=0.5*mass*rz^2 kg*m^2  num_ports=foundation.enum.numPorts2.one  w_specify=on  w_priority=High  w=0 rad/s  w_nominal_specify=off  w_nominal_value=1  w_nominal_unit=rad/s  t_specify=off  t_priority=None  t=0 N*m  t_nominal_specify=off  t_nominal_value=1  t_nominal_unit=N*m
  Memory3 : Memory
  Mode Judge : Subsystem
  Multiport Switch : MultiPortSwitch  SaturateOnIntegerOverflow=off  InputSameDT=off
  Speed Sensor : Subsystem  mask(Speed Sensor){}
      mask help: The speed unit is r/min.
  Steering Resistance : Subsystem
  Sum1 : Sum  Inputs=++++
  Tire Radius1 : Gain  Gain=-rz
  Tire Radius2 : Gain  Gain=rz
  Tire Radius3 : Gain  Gain=0
  Tire Radius4 : Gain  Gain=0.5
  Torque Actuator : Subsystem  mask(Torque Actuator){}
      mask help: The torque unit is Nm.
  Torque Sensor : Subsystem  mask(Torque Sensor){}
      mask help: The torque unit is Nm.
  Wind Resistance : Subsystem
  shaft : PMIOPort  Side=Left
  vehicle speed : Outport
  Driving Torque : Outport  Port=2
  Tf : Outport  Port=3
  wires:
  Memory3/1 -> Mode Judge/1(v)
  Grade Resistance/1(Fg) -> Sum1/3
  Steering Resistance/1(Fs) -> Sum1/4
  Tire Radius4/1 -> Add/1
  Wind Resistance/1(Fw) -> Sum1/1
  Ground Resistance/1(Ff) -> Sum1/2
  Speed Sensor/1(r/min) -> 2/1
  brake force/1 -> Tire Radius4/1
  2/1 -> vehicle speed/1, Memory3/1
  Sum1/1 -> Add/2
  Torque Sensor/1(Nm) -> 1/1
  1/1 -> Driving Torque/1
  Mode Judge/1(F) -> Multiport Switch/1
  Tire Radius2/1 -> Multiport Switch/2
  Tire Radius1/1 -> Multiport Switch/3
  Add/1 -> Tire Radius2/1, Tire Radius1/1, Tire Radius3/1
  Tire Radius3/1 -> Multiport Switch/4
  Multiport Switch/1 -> Torque Actuator/1(torque), Tf/1
  angle/1 -> Ground Resistance/2(angle), Grade Resistance/1(angle)
  fg/1 -> Ground Resistance/1(fg)
  connections:
  Torque Sensor/LConn1 -- Torque Actuator/RConn1 -- Inertia1/LConn1
  Torque Sensor/RConn1 -- Speed Sensor/LConn1 -- shaft/RConn1

== system EMT/engine/Engine/Speed Sensor ==
  Ideal Rotational Motion Sensor : fl_lib/Mechanical/Mechanical Sensors/Ideal Rotational Motion Sensor  reference=foundation.enum.MeasurementReference.difference  acceleration_port=false  velocity_port=true  position_port=true  wrap_angle=false  offset=0 rad
  PS-Simulink Converter : nesl_utility/PS-Simulink Converter  PhysicalDomain=network_engine_domain  SubClassName=ps_output  LeftPortType=input  RightPortType=output  PseudoPeriodic=off  Frequencies=[]  VectorFormat=1-D array  Unit=rad/s  AffineConversion=off
  Reference : fl_lib/Mechanical/Rotational Elements/Mechanical Rotational Reference
  Tire Radius2 : Gain  Gain=30/pi
  shaft : PMIOPort  Side=Left
  r/min : Outport
  wires:
  Tire Radius2/1 -> r/min/1
  PS-Simulink Converter/1 -> Tire Radius2/1
  connections:
  shaft/RConn1 -- Ideal Rotational Motion Sensor/LConn1
  Reference/LConn1 -- Ideal Rotational Motion Sensor/RConn1
  PS-Simulink Converter/LConn1 -- Ideal Rotational Motion Sensor/RConn2

== system EMT/engine/Engine/Subsystem ==
  ne_act : Inport
  Te_com : Inport  Port=2
  switch : Inport  Port=3
  Constant1 : Constant  Value=0
  Fcn : Fcn  Expr=u*(1103-180)/1103
  Lookup Table : Lookup  InputValues=ne_map  Table=Te_max_map  SaturateOnIntegerOverflow=off
  Product : Product  RndMeth=Zero
  Saturation : Saturate  UpperLimit=max(ne_map)  LowerLimit=min(ne_map)
  Saturation Dynamic : simulink/Discontinuities/Saturation Dynamic  OutMin=[]  OutMax=[]  OutDataTypeStr=Inherit: Same as second input  OutDataType=sfix(16)  OutScaling=2^-10  DoSatur=off
  Tire Radius2 : Gain  Gain=Y_engine
  Transfer Fcn1 : TransferFcn  Denominator=[T 1]
  Te_act : Outport
  Torque : Outport  Port=2
  wires:
  Transfer Fcn1/1 -> Product/1
  switch/1 -> Product/2
  Saturation Dynamic/1 -> Transfer Fcn1/1
  Saturation/1 -> Lookup Table/1
  Lookup Table/1 -> Saturation Dynamic/1
  Constant1/1 -> Saturation Dynamic/3
  Product/1 -> Tire Radius2/1, Te_act/1
  ne_act/1 -> Saturation/1
  Te_com/1 -> Saturation Dynamic/2
  Tire Radius2/1 -> Fcn/1
  Fcn/1 -> Torque/1

== system EMT/engine/Engine/Subsystem1 ==
  ne : Inport
  Abs1 : Abs  SaturateOnIntegerOverflow=off
  Constant1 : Constant  Value=0
  Constant2 : Constant  Value=-Tef
  Constant3 : Constant  Value=-Te_start
  Constant5 : Constant  Value=Te_start
  Switch1 : Switch  Criteria=u2 > Threshold  ZeroCross=off  SaturateOnIntegerOverflow=off  InputSameDT=off
  Switch2 : Switch  Criteria=u2 > Threshold  Threshold=0.1  ZeroCross=off  SaturateOnIntegerOverflow=off  InputSameDT=off
  Switch3 : Switch  Criteria=u2 > Threshold  Threshold=10  ZeroCross=off  SaturateOnIntegerOverflow=off  InputSameDT=off
  Torque Actuator : Subsystem  mask(Torque Actuator){}
      mask help: The torque unit is Nm.
  shaft : PMIOPort  Side=Right
  wires:
  ne/1 -> Abs1/1, Switch3/2, Switch1/2
  Constant1/1 -> Switch2/3
  Switch1/1 -> Switch2/1
  Abs1/1 -> Switch2/2
  Constant3/1 -> Switch1/1
  Constant5/1 -> Switch1/3
  Constant2/1 -> Switch3/1
  Switch2/1 -> Switch3/3
  Switch3/1 -> Torque Actuator/1(torque)
  connections:
  shaft/RConn1 -- Torque Actuator/RConn1

== system EMT/engine/Engine/Torque Actuator ==
  torque : Inport
  Ideal Torque Source : fl_lib/Mechanical/Mechanical Sources/Ideal Torque Source
  Mechanical Rotational Reference : fl_lib/Mechanical/Rotational Elements/Mechanical Rotational Reference
  Simulink-PS Converter : nesl_utility/Simulink-PS Converter  PhysicalDomain=network_engine_domain  SubClassName=ps_input  LeftPortType=input  RightPortType=output  PseudoPeriodic=off  Frequencies=[]  NoiseDistribution=none  NoiseParameters=[]  Unit=N*m  AffineConversion=off  FilteringAndDerivatives=filter  SimscapeFilterOrder=1  InputFilterTimeConstant=.001  UdotUserProvided=1
  shaft : PMIOPort  Side=Right
  wires:
  torque/1 -> Simulink-PS Converter/1
  connections:
  Simulink-PS Converter/RConn1 -- Ideal Torque Source/RConn1
  Mechanical Rotational Reference/LConn1 -- Ideal Torque Source/RConn2
  shaft/RConn1 -- Ideal Torque Source/LConn1

== system EMT/motorA/Motor/Efficiency ==
  speed : Inport
  torque : Inport  Port=2
  Abs{,1..3} (4 alike) : Abs  SaturateOnIntegerOverflow=off
  Divide : Product  Inputs=/*
  Gain1 : Gain  Gain=1/9549
  Product1 : Product  RndMeth=Zero
  Product4 : Product  RndMeth=Zero
  Saturation : Saturate  UpperLimit=max(n_motor)  LowerLimit=min(n_motor)
  Saturation1 : Saturate  UpperLimit=max(T_motor)  LowerLimit=min(T_motor)
  Saturation2 : Saturate  UpperLimit=max(n_generator)  LowerLimit=min(n_generator)
  Saturation3 : Saturate  UpperLimit=max(T_generator)  LowerLimit=min(T_generator)
  Switch : Switch  SaturateOnIntegerOverflow=off  InputSameDT=off
  generator efficiency : Lookup2D  RowIndex=n_generator  ColumnIndex=T_generator  Table=eff_generator'  LookUpMeth=Interpolation-Use End Values  SaturateOnIntegerOverflow=off  InputSameDT=off
  motor efficiency : Lookup2D  RowIndex=n_motor  ColumnIndex=T_motor  Table=eff_motor'  LookUpMeth=Interpolation-Use End Values  SaturateOnIntegerOverflow=off  InputSameDT=off
  power : Outport
  wires:
  Abs3/1 -> Saturation3/1
  Abs2/1 -> Saturation2/1
  Abs1/1 -> Saturation1/1
  Abs/1 -> Saturation/1
  Product1/1 -> Switch/3
  generator efficiency/1 -> Product1/2
  motor efficiency/1 -> Divide/1
  Divide/1 -> Switch/1
  Saturation3/1 -> generator efficiency/2
  Saturation2/1 -> generator efficiency/1
  Saturation1/1 -> motor efficiency/2
  Saturation/1 -> motor efficiency/1
  Gain1/1 -> Switch/2, Divide/2, Product1/1
  Product4/1 -> Gain1/1
  Switch/1 -> power/1
  speed/1 -> Abs2/1, Abs/1, Product4/1
  torque/1 -> Abs3/1, Abs1/1, Product4/2

== system EMT/motorA/Motor/Electrical System ==
  power : Inport
  Constant3 : Constant  Value=interp1(SOC_map,Uoc_map,SOC0)
  Controlled Current Source1 : fl_lib/Electrical/Electrical Sources/Controlled Current Source
  Divie1 : Product  Inputs=*/
  Gain : Gain  Gain=-1000
  Memory2 : Memory  InitialCondition=interp1(SOC_map,Uoc_map,SOC0)
  PS-Simulink Converter : nesl_utility/PS-Simulink Converter  PhysicalDomain=network_engine_domain  SubClassName=ps_output  LeftPortType=input  RightPortType=output  PseudoPeriodic=off  Frequencies=[]  VectorFormat=1-D array  Unit=V  AffineConversion=off
  Simulink-PS Converter : nesl_utility/Simulink-PS Converter  PhysicalDomain=network_engine_domain  SubClassName=ps_input  LeftPortType=input  RightPortType=output  PseudoPeriodic=off  Frequencies=[]  NoiseDistribution=none  NoiseParameters=[]  Unit=A  AffineConversion=off  FilteringAndDerivatives=filter  SimscapeFilterOrder=1  InputFilterTimeConstant=.001  UdotUserProvided=1
  Switch : Switch  Criteria=u2 ~= 0  SaturateOnIntegerOverflow=off  InputSameDT=off
  Voltage Sensor : fl_lib/Electrical/Electrical Sensors/Voltage Sensor
  + mot : PMIOPort  Side=Right
  - mot : PMIOPort  Port=2  Side=Right
  voltage : Outport
  wires:
  Gain/1 -> Simulink-PS Converter/1
  Memory2/1 -> Switch/1, Switch/2
  Switch/1 -> Divie1/2
  Constant3/1 -> Switch/3
  PS-Simulink Converter/1 -> voltage/1, Memory2/1
  Divie1/1 -> Gain/1
  power/1 -> Divie1/1
  connections:
  PS-Simulink Converter/LConn1 -- Voltage Sensor/RConn1
  Voltage Sensor/LConn1 -- Controlled Current Source1/LConn1 -- + mot/RConn1
  Voltage Sensor/RConn2 -- Controlled Current Source1/RConn2 -- - mot/RConn1
  Simulink-PS Converter/RConn1 -- Controlled Current Source1/RConn1

== system EMT/motorA/Motor/Mechanical Body ==
  Tm_com : Inport
  Inertia1 : fl_lib/Mechanical/Rotational Elements/Inertia  inertia=Jm kg*m^2  num_ports=foundation.enum.numPorts2.one  w_specify=on  w_priority=High  w=0 rad/s  w_nominal_specify=off  w_nominal_value=1  w_nominal_unit=rad/s  t_specify=off  t_priority=None  t=0 N*m  t_nominal_specify=off  t_nominal_value=1  t_nominal_unit=N*m
  Max & Min Torque Control : Subsystem
  Memory2 : Memory
  Resistance : Subsystem
  Speed Sensor : Subsystem  mask(Speed Sensor){}
      mask help: The speed unit is r/min.
  Torque Actuator : Subsystem  mask(Torque Actuator){}
      mask help: The torque unit is Nm.
  out : PMIOPort  Side=Right
  speed : Outport
  torque : Outport  Port=2
  wires:
  Speed Sensor/1(r/min) -> Memory2/1, speed/1
  Memory2/1 -> Resistance/1(speed), Max & Min Torque Control/1(speed)
  Max & Min Torque Control/1(torque) -> Torque Actuator/1(torque), torque/1
  Tm_com/1 -> Max & Min Torque Control/2(Tm_com)
  connections:
  Inertia1/LConn1 -- Torque Actuator/RConn1 -- Resistance/RConn1 -- Speed Sensor/LConn1 -- out/RConn1

== system EMT/motorB/Motor/Efficiency ==
  speed : Inport
  torque : Inport  Port=2
  Abs{,1..3} (4 alike) : Abs  SaturateOnIntegerOverflow=off
  Divide : Product  Inputs=/*
  Gain1 : Gain  Gain=1/9549
  Product1 : Product  RndMeth=Zero
  Product4 : Product  RndMeth=Zero
  Saturation : Saturate  UpperLimit=max(n_motor)  LowerLimit=min(n_motor)
  Saturation1 : Saturate  UpperLimit=max(T_motor)  LowerLimit=min(T_motor)
  Saturation2 : Saturate  UpperLimit=max(n_generator)  LowerLimit=min(n_generator)
  Saturation3 : Saturate  UpperLimit=max(T_generator)  LowerLimit=min(T_generator)
  Switch : Switch  SaturateOnIntegerOverflow=off  InputSameDT=off
  generator efficiency : Lookup2D  RowIndex=n_generator  ColumnIndex=T_generator  Table=eff_generator'  LookUpMeth=Interpolation-Use End Values  SaturateOnIntegerOverflow=off  InputSameDT=off
  motor efficiency : Lookup2D  RowIndex=n_motor  ColumnIndex=T_motor  Table=eff_motor'  LookUpMeth=Interpolation-Use End Values  SaturateOnIntegerOverflow=off  InputSameDT=off
  power : Outport
  wires:
  Abs3/1 -> Saturation3/1
  Abs2/1 -> Saturation2/1
  Abs1/1 -> Saturation1/1
  Abs/1 -> Saturation/1
  Product1/1 -> Switch/3
  generator efficiency/1 -> Product1/2
  motor efficiency/1 -> Divide/1
  Divide/1 -> Switch/1
  Saturation3/1 -> generator efficiency/2
  Saturation2/1 -> generator efficiency/1
  Saturation1/1 -> motor efficiency/2
  Saturation/1 -> motor efficiency/1
  Gain1/1 -> Switch/2, Divide/2, Product1/1
  Product4/1 -> Gain1/1
  Switch/1 -> power/1
  speed/1 -> Abs2/1, Abs/1, Product4/1
  torque/1 -> Abs3/1, Abs1/1, Product4/2

== system EMT/motorB/Motor/Electrical System ==
  power : Inport
  Constant3 : Constant  Value=interp1(SOC_map,Uoc_map,SOC0)
  Controlled Current Source1 : fl_lib/Electrical/Electrical Sources/Controlled Current Source
  Divie1 : Product  Inputs=*/
  Gain : Gain  Gain=-1000
  Memory2 : Memory  InitialCondition=interp1(SOC_map,Uoc_map,SOC0)
  PS-Simulink Converter : nesl_utility/PS-Simulink Converter  PhysicalDomain=network_engine_domain  SubClassName=ps_output  LeftPortType=input  RightPortType=output  PseudoPeriodic=off  Frequencies=[]  VectorFormat=1-D array  Unit=V  AffineConversion=off
  Simulink-PS Converter : nesl_utility/Simulink-PS Converter  PhysicalDomain=network_engine_domain  SubClassName=ps_input  LeftPortType=input  RightPortType=output  PseudoPeriodic=off  Frequencies=[]  NoiseDistribution=none  NoiseParameters=[]  Unit=A  AffineConversion=off  FilteringAndDerivatives=filter  SimscapeFilterOrder=1  InputFilterTimeConstant=.001  UdotUserProvided=1
  Switch : Switch  Criteria=u2 ~= 0  SaturateOnIntegerOverflow=off  InputSameDT=off
  Voltage Sensor : fl_lib/Electrical/Electrical Sensors/Voltage Sensor
  + mot : PMIOPort  Side=Right
  - mot : PMIOPort  Port=2  Side=Right
  voltage : Outport
  wires:
  Gain/1 -> Simulink-PS Converter/1
  Memory2/1 -> Switch/1, Switch/2
  Switch/1 -> Divie1/2
  Constant3/1 -> Switch/3
  PS-Simulink Converter/1 -> voltage/1, Memory2/1
  Divie1/1 -> Gain/1
  power/1 -> Divie1/1
  connections:
  PS-Simulink Converter/LConn1 -- Voltage Sensor/RConn1
  Voltage Sensor/LConn1 -- Controlled Current Source1/LConn1 -- + mot/RConn1
  Voltage Sensor/RConn2 -- Controlled Current Source1/RConn2 -- - mot/RConn1
  Simulink-PS Converter/RConn1 -- Controlled Current Source1/RConn1

== system EMT/motorB/Motor/Mechanical Body ==
  Tm_com : Inport
  Inertia1 : fl_lib/Mechanical/Rotational Elements/Inertia  inertia=Jm kg*m^2  num_ports=foundation.enum.numPorts2.one  w_specify=on  w_priority=High  w=0 rad/s  w_nominal_specify=off  w_nominal_value=1  w_nominal_unit=rad/s  t_specify=off  t_priority=None  t=0 N*m  t_nominal_specify=off  t_nominal_value=1  t_nominal_unit=N*m
  Max & Min Speed Control : Subsystem
  Memory2 : Memory
  Resistance : Subsystem
  Speed Sensor : Subsystem  mask(Speed Sensor){}
      mask help: The speed unit is r/min.
  Torque Actuator : Subsystem  mask(Torque Actuator){}
      mask help: The torque unit is Nm.
  out : PMIOPort  Side=Right
  speed : Outport
  torque : Outport  Port=2
  wires:
  Speed Sensor/1(r/min) -> Memory2/1, speed/1
  Tm_com/1 -> Max & Min Speed Control/2(Tm_com)
  Memory2/1 -> Resistance/1(speed), Max & Min Speed Control/1(speed)
  Max & Min Speed Control/1(torque) -> Torque Actuator/1(torque), torque/1
  connections:
  Speed Sensor/LConn1 -- out/RConn1 -- Torque Actuator/RConn1 -- Inertia1/LConn1 -- Resistance/RConn1

== system EMT/Control Unit/Control/EVT1_H Stage/brack force ==
  Fb_com : Outport
  wires:
  [Fb_ref] -> Fb_com/1

== system EMT/Control Unit/Control/EVT1_H Stage/clutches condition ==
  Mux2 : Mux
  Subsystem : Subsystem
  Subsystem1 : Subsystem
  Subsystem2 : Subsystem
  Subsystem4 : Subsystem
  clutch_com : Outport
  wires:
  Subsystem/1(C0) -> Mux2/1
  Subsystem2/1(C1) -> Mux2/4
  Subsystem1/1(Z2) -> Mux2/3
  Subsystem4/1(Z1) -> Mux2/2
  Mux2/1 -> clutch_com/1

== system EMT/Control Unit/Control/EVT1_H Stage/engine swich ==
  Constant1 : Constant
  engine_swich : Outport
  wires:
  Constant1/1 -> engine_swich/1

== system EMT/Control Unit/Control/EVT1_H Stage/engine torque ==
  Subsystem1 : Subsystem
  Te_com : Outport
  wires:
  [ne_act] -> Subsystem1/2(ne_act)
  [Te_ref] -> Subsystem1/1(Te_ref)
  Subsystem1/1(Te_com) -> Te_com/1

== system EMT/Control Unit/Control/EVT1_H Stage/motorA torque ==
  TA_com : Outport
  wires:
  [TA_ref] -> TA_com/1

== system EMT/Control Unit/Control/EVT1_H Stage/motorB torque ==
  TB_com : Outport
  wires:
  [TB_ref] -> TB_com/1

== system EMT/Control Unit/Control/EVT1_H Stage/motorZ torque ==
  TZ_com : Outport
  wires:
  [TZ_ref] -> TZ_com/1

== system EMT/Control Unit/Control/EVT2 Stage/brack force ==
  Fb_com : Outport
  wires:
  [Fb_ref] -> Fb_com/1

== system EMT/Control Unit/Control/EVT2 Stage/clutches condition ==
  Mux2 : Mux
  Subsystem : Subsystem
  Subsystem1 : Subsystem
  Subsystem2 : Subsystem
  Subsystem4 : Subsystem
  clutch_com : Outport
  wires:
  Mux2/1 -> clutch_com/1
  Subsystem4/1(Z1) -> Mux2/2
  Subsystem1/1(Z2) -> Mux2/3
  Subsystem2/1(C1) -> Mux2/4
  Subsystem/1(C0) -> Mux2/1

== system EMT/Control Unit/Control/EVT2 Stage/engine swich ==
  Constant1 : Constant
  engine_swich : Outport
  wires:
  Constant1/1 -> engine_swich/1

== system EMT/Control Unit/Control/EVT2 Stage/engine torque ==
  Te_com : Outport
  wires:
  [Te_ref] -> Te_com/1

== system EMT/Control Unit/Control/EVT2 Stage/motorA torque ==
  TA_com : Outport
  wires:
  [TA_ref] -> TA_com/1

== system EMT/Control Unit/Control/EVT2 Stage/motorB torque ==
  TB_com : Outport
  wires:
  [TB_ref] -> TB_com/1

== system EMT/Control Unit/Control/EVT2 Stage/motorZ torque ==
  Lookup Table : Lookup  InputValues=nZ_map  Table=TZ_max_map  SaturateOnIntegerOverflow=off
  Lookup Table1 : Lookup  InputValues=nZ_map  Table=TZ_min_map  SaturateOnIntegerOverflow=off
  Saturation Dynamic : simulink/Discontinuities/Saturation Dynamic  OutMin=[]  OutMax=[]  OutDataTypeStr=Inherit: Same as second input  OutDataType=sfix(16)  OutScaling=2^-10  DoSatur=off
  Saturation1 : Saturate  UpperLimit=max(nZ_map)  LowerLimit=min(nZ_map)
  Saturation2 : Saturate  UpperLimit=max(nZ_map)  LowerLimit=min(nZ_map)
  Subsystem1 : Subsystem
  TZ_com : Outport
  wires:
  Saturation Dynamic/1 -> TZ_com/1
  [nZ_act] -> Saturation1/1, Saturation2/1, Subsystem1/1(nZ_act)
  Lookup Table/1 -> Saturation Dynamic/1
  Lookup Table1/1 -> Saturation Dynamic/3
  Saturation1/1 -> Lookup Table/1
  Saturation2/1 -> Lookup Table1/1
  Subsystem1/1(TZ_com) -> Saturation Dynamic/2

== system EMT/Control Unit/Control/Power Distribution/Electric Power Requirement ==
  Voltage : Inport
  SOC : Inport  Port=2
  ElectricPower : Inport  Port=3
  1-D Lookup Table : Lookup_n-D  NumberOfTableDimensions=1  BreakpointsForDimension1=SOC_epr  Table=Pb_epr  RndMeth=Simplest
  1-D Lookup Table2 : Lookup_n-D  NumberOfTableDimensions=1  BreakpointsForDimension1=Voltage_epr  Table=Pb_max  RndMeth=Simplest
  1-D Lookup Table3 : Lookup_n-D  NumberOfTableDimensions=1  BreakpointsForDimension1=Voltage_epr  Table=Pb_min  RndMeth=Simplest
  Add : Sum  Inputs=+--
  Constant : Constant  Value=PN0
  Data : Subsystem
  Memory3 : Memory  InitialCondition=SOC0
  Memory7 : Memory  InitialCondition=SOC0
  Mux : Mux
  PZ_com : Constant  Value=0
  Saturation1 : Saturate  UpperLimit=max(SOC_epr)  LowerLimit=min(SOC_epr)
  Saturation2 : Saturate  UpperLimit=max(Voltage_epr)  LowerLimit=min(Voltage_epr)
  PN_k : Outport
  wires:
  1-D Lookup Table2/1 -> Data/2(PN_max), Mux/2
  1-D Lookup Table3/1 -> Data/3(PN_min), Mux/3
  Saturation2/1 -> 1-D Lookup Table3/1, 1-D Lookup Table2/1
  Voltage/1 -> Memory7/1
  Saturation1/1 -> 1-D Lookup Table/1
  Add/1 -> Data/1(PN_com), Mux/1
  1-D Lookup Table/1 -> Add/1
  Memory3/1 -> Saturation1/1
  SOC/1 -> Memory3/1
  Mux/1 -> PN_k/1
  Memory7/1 -> Saturation2/1
  Constant/1 -> Add/3
  ElectricPower/1 -> Add/2
  PZ_com/1 -> Mux/4
